simulink model "CruiseControlPID"  (R2024b)
settings: Solver=VariableStepAuto  StartTime=0.0  StopTime=10.0  RelTol=1e-3
model workspace (MAT data in the model file):
  Cd = 1
  Kd = 1
  Ki = 1
  Km = 1
  Kp = 1
  c = 1
  m = 1
  mu = 1
  test = 3
  theta = 0
  v_des = 30
settings Model: Creator=andre  LastModifiedBy=andre

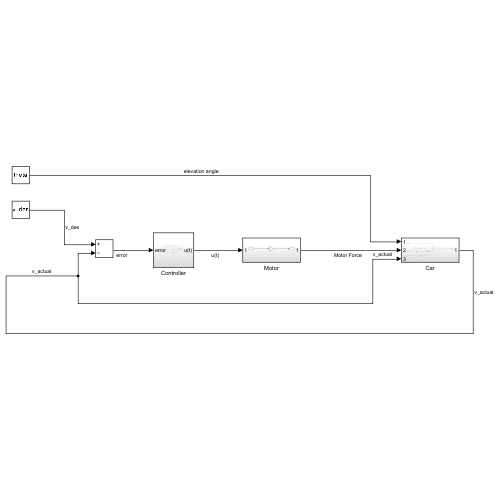
[thumbnail: Simulink's stored preview of the top-level diagram]
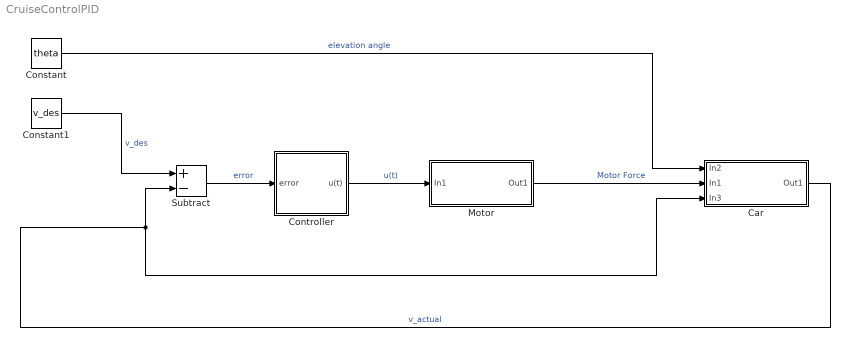
== system CruiseControlPID ==
  Car : Subsystem
  Constant : Constant  Value=theta
  Constant1 : Constant  Value=v_des
  Controller : Subsystem
  Motor : Subsystem
  Subtract : Sum  Inputs=+-
  wires:
  Constant1/1 -> Subtract/1  "v_des"
  Motor/1(Out1) -> Car/2(In1)  "Motor Force"
  Constant/1 -> Car/1(In2)  "elevation angle"
  Car/1(Out1) -> Subtract/2, Car/3(In3)  "v_actual"
  Subtract/1 -> Controller/1(error)  "error"
  Controller/1(u(t)) -> Motor/1(In1)  "u(t)"

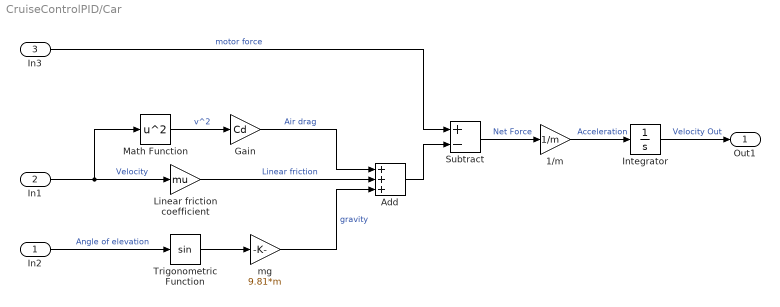
== system CruiseControlPID/Car ==
  In2 : Inport
  In1 : Inport  Port=2
  In3 : Inport  Port=3
  1/m : Gain  Gain=1/m
  Add : Sum  Inputs=+++
  Gain : Gain  Gain=Cd
  Integrator : Integrator
  Linear friction coefficient : Gain  Gain=mu
  Math Function : Math  Operator=square
  Subtract : Sum  Inputs=+-
  Trigonometric Function : Trigonometry
  mg : Gain  Gain=9.81*m
  Out1 : Outport
  wires:
  In1/1 -> Math Function/1, Linear friction coefficient/1  "Velocity"
  Linear friction coefficient/1 -> Add/2  "Linear friction"
  Math Function/1 -> Gain/1  "v^2"
  In2/1 -> Trigonometric Function/1  "Angle of elevation"
  Trigonometric Function/1 -> mg/1
  mg/1 -> Add/3  "gravity"
  Gain/1 -> Add/1  "Air drag"
  In3/1 -> Subtract/1  "motor force"
  Add/1 -> Subtract/2
  Subtract/1 -> 1/m/1  "Net Force"
  Integrator/1 -> Out1/1  "Velocity Out"
  1/m/1 -> Integrator/1  "Acceleration"

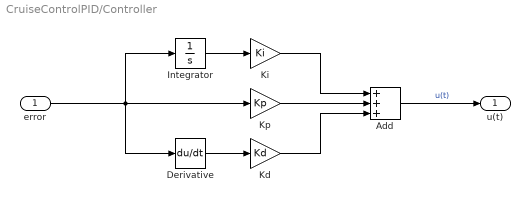
== system CruiseControlPID/Controller ==
  error : Inport
  Add : Sum  Inputs=+++
  Derivative : Derivative
  Integrator : Integrator
  Kd : Gain  Gain=Kd
  Ki : Gain  Gain=Ki
  Kp : Gain  Gain=Kp
  u(t) : Outport
  wires:
  Kp/1 -> Add/2
  error/1 -> Kp/1, Integrator/1, Derivative/1
  Add/1 -> u(t)/1  "u(t)"
  Integrator/1 -> Ki/1
  Derivative/1 -> Kd/1
  Ki/1 -> Add/1
  Kd/1 -> Add/3

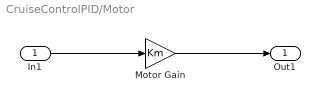
== system CruiseControlPID/Motor ==
  In1 : Inport
  Motor Gain : Gain  Gain=Km
  Out1 : Outport
  wires:
  In1/1 -> Motor Gain/1
  Motor Gain/1 -> Out1/1
